simulink model "eVTOL_R2023b"  (R2023b)
settings: Solver=ode4  StartTime=0.0  StopTime=10  FixedStep=0.005  RelTol=1e-3
InitFcn:
  | addpath(fileparts(get_param(bdroot,'FileName')));
  | sub = [bdroot '/Trajectory Generator'];
  | mode = str2double(get_param([bdroot '/Trajectory Mode'],'Value'));
  | assert(ismember(mode,[1 2]),'Mode must be 1 (SP) or 2 (circle).');
  | if mode == 1
  |  start = str2num(get_param([sub '/Start Position'],'Value'));
  |  initial = [start(1);0;start(2);0;0;0];
  | else
  |  center = str2num(get_param([sub '/Circle Center'],'Value'));
  |  R = str2double(get_param([sub '/Circle Radius'],'Value'));
  |  T = str2double(get_param([sub '/Circle Period'],'Value'));
  |  w = 0; if T > 0, w = 2*pi/T; end
  |  q = [-R*w^2;1]; dq = [0;-R*w^3];
  |  assert(q.'*q>0.05^2,'Initial thrust is singular.');
  |  omega = (q(1)*dq(2)-q(2)*dq(1))/(q.'*q);
  |  initial = [center(1)+R;0;center(2);R*w;atan2(-q(1),q(2));omega];
  | end
  | set_param([bdroot '/VTOL Plant/Six-State Integrator'],'InitialCondition',mat2str(initial,17));
StopFcn:
  | schedule_evtol_plot;
model workspace (MAT data in the model file):
  param.g = 1
settings Model: Creator=aljunaidazme  LastModifiedBy=aljunaidazme
settings DataIOCC: ReturnWorkspaceOutputs=off
settings ModelReferenceCC: UpdateModelReferenceTargets=IfOutOfDate
settings SFSimCC: SimGPUStackLimitPerThread=51200
settings RTWCC: GPUStackLimitPerThread=51200  GPUComputeCapability=7.5
settings ConfigComp: CovMetricSettings=de  CovBoundaryAbsTol=1.0e-5

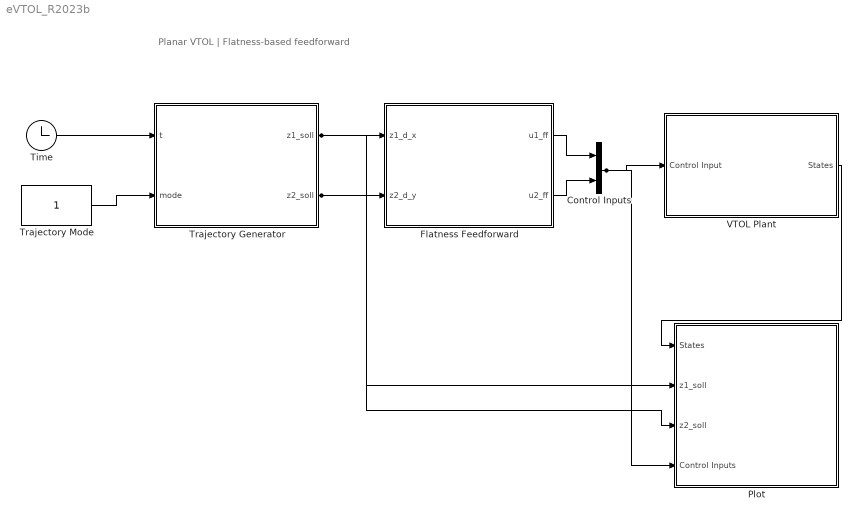
== system eVTOL_R2023b ==
  note: Planar VTOL | Flatness-based feedforward
  Control Inputs : Mux  Inputs=2
  Flatness Feedforward : Subsystem
  Plot : Subsystem
  Time : Clock
  Trajectory Generator : Subsystem
  Trajectory Mode : Constant
  VTOL Plant : Subsystem
  wires:
  Time/1 -> Trajectory Generator/1(t)
  Trajectory Mode/1 -> Trajectory Generator/2(mode)
  Trajectory Generator/1(z1_soll) -> Flatness Feedforward/1(z1_d_x), Plot/2(z1_soll)
  Trajectory Generator/2(z2_soll) -> Flatness Feedforward/2(z2_d_y), Plot/3(z2_soll)
  Flatness Feedforward/1(u1_ff) -> Control Inputs/1
  Flatness Feedforward/2(u2_ff) -> Control Inputs/2
  Control Inputs/1 -> VTOL Plant/1(Control Input), Plot/4(Control Inputs)
  VTOL Plant/1(States) -> Plot/1(States)

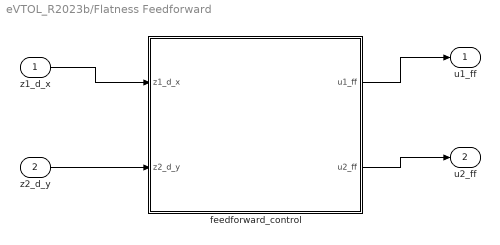
== system eVTOL_R2023b/Flatness Feedforward ==
  z1_d_x : Inport
  z2_d_y : Inport  Port=2
  feedforward_control : MATLAB Function  TreatAsAtomicUnit=on
  u1_ff : Outport
  u2_ff : Outport  Port=2
  wires:
  z1_d_x/1 -> feedforward_control/1(z1_d_x)
  feedforward_control/1(u1_ff) -> u1_ff/1
  z2_d_y/1 -> feedforward_control/2(z2_d_y)
  feedforward_control/2(u2_ff) -> u2_ff/1

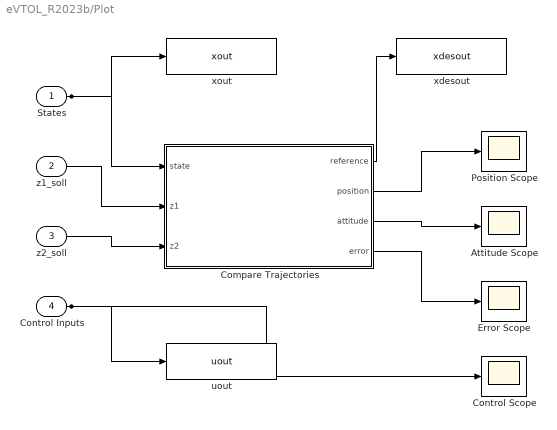
== system eVTOL_R2023b/Plot ==
  States : Inport
  z1_soll : Inport  Port=2
  z2_soll : Inport  Port=3
  Control Inputs : Inport  Port=4
  Attitude Scope : Scope
  Compare Trajectories : MATLAB Function  TreatAsAtomicUnit=on
  Control Scope : Scope
  Error Scope : Scope
  Position Scope : Scope
  uout : ToWorkspace  VariableName=uout  SaveFormat=Timeseries  SampleTime=-1
  xdesout : ToWorkspace  VariableName=xdesout  SaveFormat=Timeseries  SampleTime=-1
  xout : ToWorkspace  VariableName=xout  SaveFormat=Timeseries  SampleTime=-1
  wires:
  States/1 -> Compare Trajectories/1(state), xout/1
  z1_soll/1 -> Compare Trajectories/2(z1)
  z2_soll/1 -> Compare Trajectories/3(z2)
  Compare Trajectories/2(position) -> Position Scope/1
  Compare Trajectories/3(attitude) -> Attitude Scope/1
  Compare Trajectories/4(error) -> Error Scope/1
  Control Inputs/1 -> Control Scope/1, uout/1
  Compare Trajectories/1(reference) -> xdesout/1

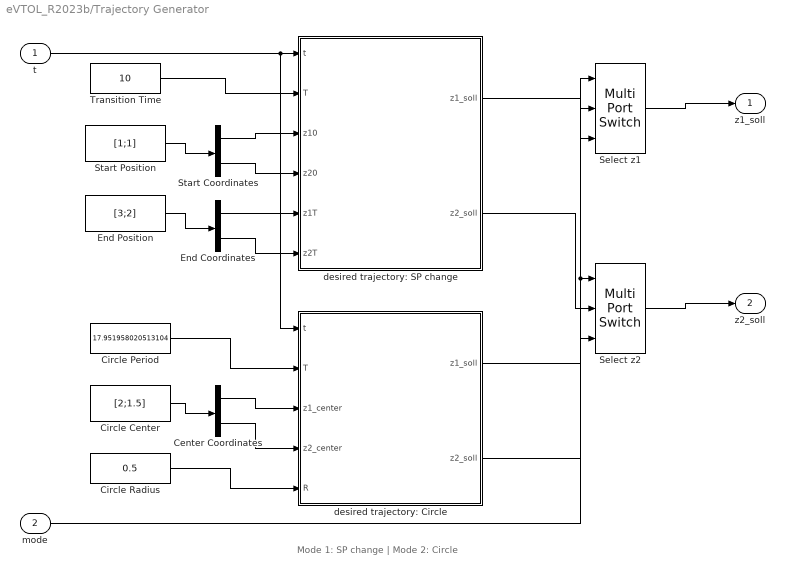
== system eVTOL_R2023b/Trajectory Generator ==
  note: Mode 1: SP change | Mode 2: Circle
  t : Inport
  mode : Inport  Port=2
  Center Coordinates : Demux  Outputs=2
  Circle Center : Constant  Value=[2;1.5]
  Circle Period : Constant  Value=17.951958020513104
  Circle Radius : Constant  Value=0.5
  End Coordinates : Demux  Outputs=2
  End Position : Constant  Value=[3;2]
  Select z1 : MultiPortSwitch  Inputs=2  SaturateOnIntegerOverflow=off  InputSameDT=off
  Select z2 : MultiPortSwitch  Inputs=2  SaturateOnIntegerOverflow=off  InputSameDT=off
  Start Coordinates : Demux  Outputs=2
  Start Position : Constant  Value=[1;1]
  Transition Time : Constant  Value=10
  desired trajectory: Circle : MATLAB Function  TreatAsAtomicUnit=on
  desired trajectory: SP change : MATLAB Function  TreatAsAtomicUnit=on
  z1_soll : Outport
  z2_soll : Outport  Port=2
  wires:
  t/1 -> desired trajectory: SP change/1(t), desired trajectory: Circle/1(t)
  Transition Time/1 -> desired trajectory: SP change/2(T)
  Start Position/1 -> Start Coordinates/1
  End Position/1 -> End Coordinates/1
  Start Coordinates/1 -> desired trajectory: SP change/3(z10)
  End Coordinates/1 -> desired trajectory: SP change/5(z1T)
  Start Coordinates/2 -> desired trajectory: SP change/4(z20)
  End Coordinates/2 -> desired trajectory: SP change/6(z2T)
  Circle Period/1 -> desired trajectory: Circle/2(T)
  Circle Center/1 -> Center Coordinates/1
  Center Coordinates/1 -> desired trajectory: Circle/3(z1_center)
  Center Coordinates/2 -> desired trajectory: Circle/4(z2_center)
  Circle Radius/1 -> desired trajectory: Circle/5(R)
  mode/1 -> Select z1/1, Select z2/1
  desired trajectory: SP change/1(z1_soll) -> Select z1/2
  desired trajectory: Circle/1(z1_soll) -> Select z1/3
  Select z1/1 -> z1_soll/1
  desired trajectory: SP change/2(z2_soll) -> Select z2/2
  desired trajectory: Circle/2(z2_soll) -> Select z2/3
  Select z2/1 -> z2_soll/1

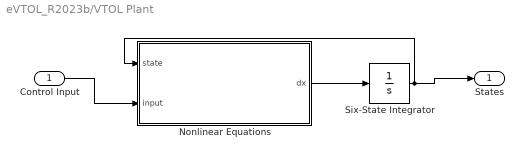
== system eVTOL_R2023b/VTOL Plant ==
  Control Input : Inport
  Nonlinear Equations : MATLAB Function  TreatAsAtomicUnit=on
  Six-State Integrator : Integrator  InitialCondition=[1;0;1;0;0;0]
  States : Outport
  wires:
  Control Input/1 -> Nonlinear Equations/2(input)
  Nonlinear Equations/1(dx) -> Six-State Integrator/1
  Six-State Integrator/1 -> States/1, Nonlinear Equations/1(state)

== matlab function eVTOL_R2023b/Trajectory Generator/desired trajectory: SP change ==
  data: t input; z1_soll output; T input; z10 input; z20 input; z1T input; z2T input; z2_soll output
function [z1_soll, z2_soll] = fcn(t, T, z10, z20, z1T, z2T)
if T > 0
    tau = min(max(t/T,0),1);
    % Polynomial (C^4 smooth)
    P  = 126*tau^5 - 420*tau^6 + 540*tau^7 - 315*tau^8 + 70*tau^9;
    dP = (630*tau^4 - 2520*tau^5 + 3780*tau^6 - 2520*tau^7 + 630*tau^8) / T;
    d2P = (2520*tau^3 - 12600*tau^4 + 22680*tau^5 - 17640*tau^6 + 5040*tau^7) / T^2;
    d3P = (7560*tau^2 - 50400*tau^3 + 113400*tau^4 - 105840*tau^5 + 35280*tau^6) / T^3;
    d4P = (15120*tau - 151200*tau^2 + 453600*tau^3 - 529200*tau^4 + 211680*tau^5) / T^4;
else
    % Hold initial state if T <= 0.
    P = 0; dP = 0; d2P = 0; d3P = 0; d4P = 0;
end
% z1 trajectory
z1 = z10 + (z1T - z10) * P;
dz1 = (z1T - z10) * dP;
d2z1 = (z1T - z10) * d2P;
d3z1 = (z1T - z10) * d3P;
d4z1 = (z1T - z10) * d4P;
% z2 trajectory
z2 = z20 + (z2T - z20) * P;
dz2 = (z2T - z20) * dP;
d2z2 = (z2T - z20) * d2P;
d3z2 = (z2T - z20) * d3P;
d4z2 = (z2T - z20) * d4P;
z1_soll = [z1; dz1; d2z1; d3z1; d4z1];
z2_soll = [z2; dz2; d2z2; d3z2; d4z2];
end

== matlab function eVTOL_R2023b/VTOL Plant/Nonlinear Equations ==
  data: state input; dx output; input input
function dx = dynamics(state, input)
% State order: [x; vx; y; vy; theta; omega].
% Input order: [normalized thrust; angular acceleration].
dx = zeros(6,1);
dx(1) = state(2);
dx(2) = -input(1)*sin(state(5));
dx(3) = state(4);
dx(4) = input(1)*cos(state(5))-1;
dx(5) = state(6);
dx(6) = input(2);
end

== matlab function eVTOL_R2023b/Flatness Feedforward/feedforward_control ==
  data: z1_d_x input; u1_ff output; z2_d_y input; u2_ff output; param parameter
function [u1_ff, u2_ff] = feedforward_control(z1_d_x, z2_d_y, param)
% Flatness-based feedforward control for the normalized planar VTOL.

% Parameters: g = 1 for the exercise's normalized plant.
g = param.g;

% Unpack z1* derivatives: [z1; dz1; d2z1; d3z1; d4z1].
z1   = z1_d_x(1);
dz1  = z1_d_x(2);
d2z1 = z1_d_x(3);
d3z1 = z1_d_x(4);
d4z1 = z1_d_x(5);

% Unpack z2* derivatives: [z2; dz2; d2z2; d3z2; d4z2].
z2   = z2_d_y(1);
dz2  = z2_d_y(2);
d2z2 = z2_d_y(3);
d3z2 = z2_d_y(4);
d4z2 = z2_d_y(5);

% Position and velocity are unpacked for clarity; these inputs depend on
% acceleration, jerk and snap. A near-zero thrust makes inversion singular.
den = d2z1^2 + (d2z2 + g)^2;
assert(den > 0.05^2);

% VTOL thrust magnitude.
u1_ff = sqrt(den);

% VTOL angular acceleration: second time derivative of desired attitude.
u2_ff = 2*(d2z1*d3z1 + (d2z2 + g)*d3z2) ...
    *(d3z1*(d2z2 + g) - d2z1*d3z2)/den^2 ...
    - (d4z1*(d2z2 + g) - d2z1*d4z2)/den;
end

== matlab function eVTOL_R2023b/Plot/Compare Trajectories ==
  data: state input; reference output; z1 input; z2 input; position output; attitude output; error output
function [reference,position,attitude,error] = compare(state,z1,z2)
reference = [z1.';z2.'];
position = [state(1);z1(1);state(3);z2(1)];
den = z1(3)^2+(z2(3)+1)^2;
theta = atan2(-z1(3),z2(3)+1);
omega = (z1(3)*z2(4)-(z2(3)+1)*z1(4))/den;
attitude = [state(5);theta;state(6);omega];
error = [state(1)-z1(1);state(3)-z2(1)];
end

== matlab function eVTOL_R2023b/Trajectory Generator/desired trajectory: Circle ==
  data: t input; z1_soll output; T input; z1_center input; z2_center input; R input; z2_soll output
function [z1_soll, z2_soll] = fcn(t, T, z1_center, z2_center, R)
% T is the time for one revolution; center coordinates are not initial position.
if T > 0
    w = 2*pi/T;
else
    w = 0;
end
z1 = z1_center + R*cos(w*t);
dz1 = -R*w*sin(w*t);
d2z1 = -R*w^2*cos(w*t);
d3z1 = R*w^3*sin(w*t);
d4z1 = R*w^4*cos(w*t);

z2 = z2_center + R*sin(w*t);
dz2 = R*w*cos(w*t);
d2z2 = -R*w^2*sin(w*t);
d3z2 = -R*w^3*cos(w*t);
d4z2 = R*w^4*sin(w*t);
z1_soll = [z1; dz1; d2z1; d3z1; d4z1];
z2_soll = [z2; dz2; d2z2; d3z2; d4z2];
end
